simulink model "MIMO_BPSK_Alamouti_USRPTx"  (R2026a)
settings: Solver=FixedStepDiscrete  StopTime=inf
PreLoadFcn:
  | PayloadBitRate = 250e3/4
  | 
  | EbNo = 15;
  | 
  | barker=[+1 +1 +1 +1 +1 -1 -1 +1 +1 -1 +1 -1 +1].' > 0;
  | hModulator = comm.BPSKModulator;
  | hModulator.PhaseOffset = 0;
  | modHeader = step(hModulator, barker);
model workspace: external: MAT-File modelspace.mat (data not in the file)
undefined symbols (not defined in the file or in its folder): gcbh, rcfiltgaincompat
libraries: commmimo x1, commdigbbndpm3 x1, commfilt2 x1, commsdrhw_v2 x1
settings Model: LastModifiedBy=dawn
settings DataIOCC: SignalLoggingSaveFormat=ModelDataLogs
settings DebuggingCC: UnderspecifiedInitializationDetection=Classic
settings HardwareCC: ProdHWDeviceType=32-bit Generic
settings GRTTargetCC: CombineOutputUpdateFcns=off  GRTInterface=on

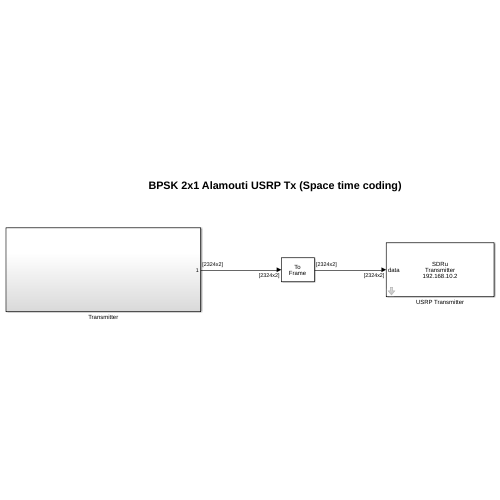
[thumbnail: Simulink's stored preview of the top-level diagram]
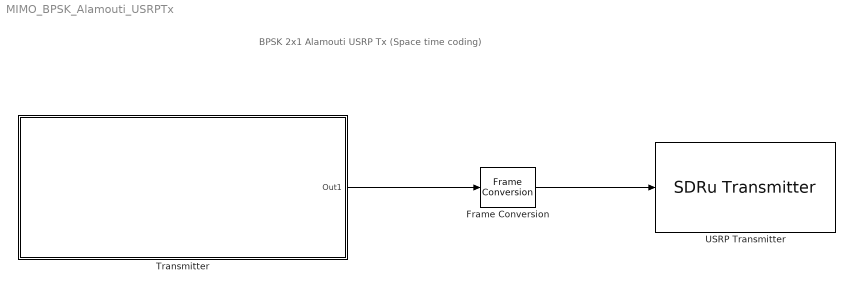
== system MIMO_BPSK_Alamouti_USRPTx ==
  note: BPSK 2x1 Alamouti USRP Tx (Space time coding)
  Frame Conversion : FrameConversion
  Transmitter : Subsystem
  USRP Transmitter : commsdrhw_v2/SDRu Transmitter  rxtx=tx  initializeIPAddress=0  devMap=0  USRP2_IP=192.168.10.2  USRP_IP_X300=192.168.10.2  USRP_IP_X310=192.168.10.2  USRP_IP_N300=No devices found  USRP_IP_N310=192.168.10.2  USRP_IP_N320=No devices found  USRP_IP_E320=No devices found  USRP_IP_X410=No devices found  USRP_serialNumB200=F4F58D  USRP_serialNumB210=30ECB7B  platform=X310  prevPlatform=X310  lastIPAddressPopup=192.168.10.2  USRP_ID=192.168.10.2  LastIPAddress=192.168.10.2  ChannelMapping=[1 2]  centerFrequencySrc=Dialog  centerFrequency=921e6  loOffsetSrc=Dialog  loOffset=0  gainSrc=Dialog  gain=50  PPSSource=Internal  clockSource=Internal  EnableGPSLock=off  EnsureSyncGPSTime=off  EnableTimeTrigger=off  triggerTime=5  enableMIMOCableSync=off  EnableRefLock=off  masterClkRateParam=184.32e6  masterClkRateB200=250e3  masterClkRateB210=25e6  masterClkRateX300=200e6  masterClkRateX310=184.32e6  masterClkRateN300=125e6  masterClkRateN310=125e6  masterClkRateN320=200e6  masterClkRateE320=30.72e6  masterClkRateX410=250e6  decimInterpSrc=Dialog  lastDecimSource=Dialog  decimInterp=100  USRP2_IP_NUM=[49 57 50 46 49 54 56 46 49 48 46 50]  frameLength=362  sampleRate=1843200  TransportDataType=int16  outputDatatype=Same as transport data type  overrunUnderrunPort=off  sampleTime=1  dboardInfo=|  HOST_DATA_PORT=30000  HOST_CONTROL_PORT=30001  USRP2_DATA_PORT=32769  USRP2_CONTROL_PORT=32768  bufferMode=Continuous streaming  EnableBurstMode=off  NumFramesInBurst=100
      | dbid: 0
      |           dbName: 'no db found'
      |          freqMin: 0
      |          freqMax: 0
      |          gainMin: 0
      |          gainMax: 0
      |     gainStepSize: 0
  wires:
  Transmitter/1(Out1) -> Frame Conversion/1
  Frame Conversion/1 -> USRP Transmitter/1

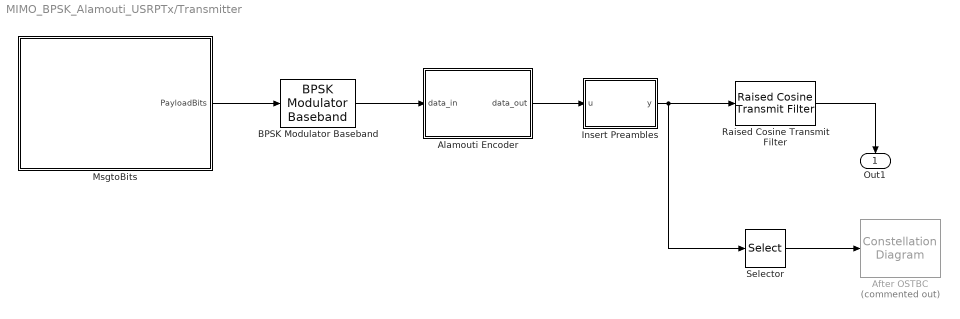
== system MIMO_BPSK_Alamouti_USRPTx/Transmitter ==
  After OSTBC : ConstellationDiagram  Tag=ScatterPlot  Commented=on  WindowPosition=[393.000000,266.000000,600.000000,600.000000,]  ScopeFrameLocation=window  SamplesPerSymbol=2  SymbolsToDisplaySource=Property  SymbolsToDisplay=1000  ReferenceConstellation=BPSK  Title=After Raised Cosine Rx Filter  XLimits=[-1.25 1.25]  YLimits=[-1.25 1.25]  AxesLimits=[-1.25 1.25]  DefaultConfigurationName=comm.scopes.ConstellationDiagramBlockCfg
  Alamouti Encoder : Subsystem  mask(Constant){Select_1=2}
      mask prompts: Select_1 "Encoder Selection"
      mask help:
      | Encoder Selection Parameter:
      | 1 Simulink Block
      | 2 User Defined Function
      mask init:
      | Select=1
  BPSK Modulator Baseband : commdigbbndpm3/BPSK Modulator Baseband  Ph=0  outDtype=double  outWordLen=16  outUDDataType=sfix(16)  outFracLenMode=Best precision  outFracLen=15  outDataTypeStr=double  outLastDataTypeStr=double
  Insert Preambles : MATLAB Function  TreatAsAtomicUnit=on
  MsgtoBits : MATLAB Function  TreatAsAtomicUnit=on
  Raised Cosine Transmit Filter : commfilt2/Raised Cosine Transmit Filter  filtType=Square root  R=0.5  filtSpan=10  N=4  filterGain=rcfiltgaincompat(gcbh)  InputProcessing=Columns as channels (frame based)  RateOptions=Enforce single-rate processing  framing=Mute  checkCoeff=off  variableName=rcTxFilt  checkGain=Normalized  sampMode=Mute  saveAsFlag=0  currentFiltSpan=10  D=(10)/2  launchFVT=off  roundingMode=Floor  overflowMode=off  coeffDataTypeStr=Inherit: Same word length as input  coeffMin=[]  coeffMax=[]  coeffLastDataTypeStr=Inherit: Same word length as input  outputDataTypeStr=Inherit: Same as accumulator  outputMin=[]  outputMax=[]  outputLastDataTypeStr=Inherit: Same as accumulator
  Selector : Selector  NumberOfDimensions=2  InputPortWidth=3  IndexOptions=Select all,Index vector (dialog)  Indices=[1 3],1  OutputSizes=1,1
  Out1 : Outport  VectorParamsAs1DForOutWhenUnconnected=off
  wires:
  Insert Preambles/1(y) -> Raised Cosine Transmit Filter/1, Selector/1
  BPSK Modulator Baseband/1 -> Alamouti Encoder/1(data_in)
  MsgtoBits/1(PayloadBits) -> BPSK Modulator Baseband/1
  Alamouti Encoder/1(data_out) -> Insert Preambles/1(u)
  Raised Cosine Transmit Filter/1 -> Out1/1
  Selector/1 -> After OSTBC/1

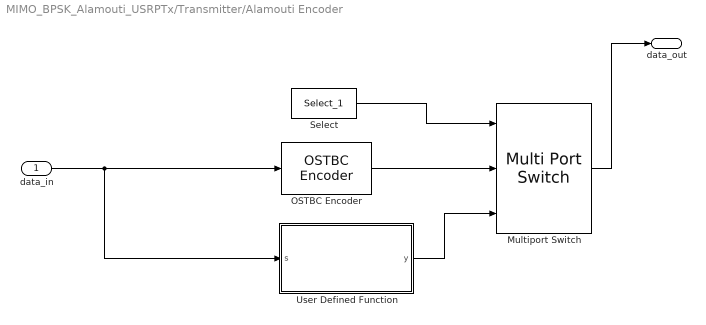
== system MIMO_BPSK_Alamouti_USRPTx/Transmitter/Alamouti Encoder ==
  data_in : Inport
  Multiport Switch : MultiPortSwitch  Inputs=2  SaturateOnIntegerOverflow=off  InputSameDT=off
  OSTBC Encoder : commmimo/OSTBC Encoder  numTx=2  rate=3/4  overflowMode=Wrap  OvFlMode=off  OvFlModeLastStrValue=off
  Select : Constant  Value=Select_1  VectorParams1D=off  OutMin=1  OutMax=5  OutDataTypeStr=Inherit: Inherit via back propagation
  "User Defined Function " : MATLAB Function  TreatAsAtomicUnit=on
  data_out : Outport  VectorParamsAs1DForOutWhenUnconnected=off
  wires:
  data_in/1 -> "User Defined Function "/1(s), OSTBC Encoder/1
  Select/1 -> Multiport Switch/1
  OSTBC Encoder/1 -> Multiport Switch/2
  "User Defined Function "/1(y) -> Multiport Switch/3
  Multiport Switch/1 -> data_out/1

== matlab function MIMO_BPSK_Alamouti_USRPTx/Transmitter/Insert Preambles ==
  data: u input; y output
function y = fcn(u)
% u: [560x2] Alamouti-coded symbols (col 1 = Ant #1, col 2 = Ant #2)
% y: [581x2] = [Barker (13) ; Pilots (8) ; Data (560)]

% Modulated Barker code (13x1), BPSK: bit 0 -> +1, bit 1 -> -1
barker = [+1 +1 +1 +1 +1 -1 -1 +1 +1 -1 +1 -1 +1].' > 0;
modBarkerCode = complex(1 - 2*double(barker));

% Orthogonal pilots (8x2)
pilots = [1 1; 1 -1; 1 1; 1 -1; 1 1; 1 -1; 1 1; 1 -1];

% Same Barker on both antennas, then pilots, then data
y = [repmat(modBarkerCode, 1, 2); pilots; u];
end

== matlab function MIMO_BPSK_Alamouti_USRPTx/Transmitter/Alamouti Encoder/User Defined Function  ==
  data: s input; y output size=[560, 2]
function y = Alamouti_encoder(s)
% s: [560x1] BPSK symbols
% y: [560x2] col 1 = Ant #1, col 2 = Ant #2
N  = length(s);
y  = complex(zeros(N, 2));

s1 = s(1:2:end);             % odd symbols
s2 = s(2:2:end);             % even symbols

y(1:2:end, 1) =  s1;         % slot t,   Ant 1
y(1:2:end, 2) =  s2;         % slot t,   Ant 2
y(2:2:end, 1) = -conj(s2);   % slot t+1, Ant 1
y(2:2:end, 2) =  conj(s1);   % slot t+1, Ant 2
end

== matlab function MIMO_BPSK_Alamouti_USRPTx/Transmitter/MsgtoBits ==
  data: PayloadBits output double size=[560, 1]
function PayloadBits   = MsgtoBits
%This function converts a message to payloadBits with padding 

%% Configuration paramters
%System Paramters
   NumBitsPerCharacter  = 7;
   
%% Alogrithm 
%Payload message
    PayloadMessage = 'Welcome to the school of electrical and information engineering, Uni. of Sydney!';
    %PayloadMessage = zeros(80,1) +127;
    
%Convert message to bits
    coder.extrinsic('dec2bin');
    msgInBits = coder.const(double(dec2bin(PayloadMessage, NumBitsPerCharacter).'));
    PayloadBits = msgInBits(:) - 48;
